simulink model "Battery_PowerEnergy_GridSOC_netz"  (R2024b)
settings: Solver=ode3  StartTime=0.0  StopTime=8759.75  FixedStep=10  RelTol=1e-3
model workspace (MAT data in the model file):
  Cc_tab = [1.5 1.55813461538 1.61558974359 1.67194230769 1.72676923077 1.7796474359 1.83015384615 1.87786538462 1.92235897436 1.96321153846 2 2.03486538462 2.07007692308 2.10540384615 2.14061538462 2.17548076923 2.20976923077 2.24325 2.27569230769 2.30686538462 2.33653846154 2.36448076923 2.39046153846 2.41425 2.43561538462 2.45432692308 2.47015384615 2.48286538462 2.49223076923 2.49801923077 2.5 2.49771933962 2.49109433962 2.4804504717 2.46611320755 2.44840801887 2.42766037736 2.40419575472 2.37833962264 2.35041745283 2.32075471698 2.28967688679 2.25750943396 2.22457783019 2.19120754717 2.1577240566 2.12445283019 2.09171933962 2.0598490566 2.02916745283 2 1.97106753319 1.94093774983 1.90970641509 1.8774692942 1.84432215234 1.81036075472 1.77568086653 1.74037825297 1.70454867925 1.66828791055 1.63169171209 1.59485584906 1.55787608665 1.52084819008 1.48386792453 1.44703105521 1.41043334731 1.37417056604 1.33833847659 1.30303284416 1.26834943396 1.23438401118 1.20123234102 1.16899018868 1.13775331936 1.10761749825 1.07867849057 1.0510320615 1.02477397624 1 0.97712 0.95616 0.93664 0.91808 0.9 0.88192 0.86336 0.84384 0.82288 0.8 0.77531 0.74928 0.72197 0.69344 0.66375 0.63296 0.60113 0.56832 0.53459 0]
  Cd_tab = [0 0.811245454545 0.824872727273 0.840718181818 0.858618181818 0.878409090909 0.899927272727 0.923009090909 0.947490909091 0.973209090909 1 1.02948863636 1.06318181818 1.10073863636 1.14181818182 1.18607954545 1.23318181818 1.28278409091 1.33454545455 1.388125 1.44318181818 1.499375 1.55636363636 1.61380681818 1.67136363636 1.72869318182 1.78545454545 1.84130681818 1.89590909091 1.94892045455 2 2.05044932432 2.1017027027 2.15361824324 2.20605405405 2.25886824324 2.31191891892 2.36506418919 2.41816216216 2.47107094595 2.52364864865 2.57575337838 2.62724324324 2.67797635135 2.72781081081 2.77660472973 2.82421621622 2.87050337838 2.91532432432 2.95853716216 3 3.04114214214 3.08337137137 3.12651351351 3.17039439439 3.21483983984 3.25967567568 3.30472772773 3.34982182182 3.39478378378 3.43943943944 3.48361461461 3.52713513514 3.56982682683 3.61151551552 3.65202702703 3.69118718719 3.72882182182 3.76475675676 3.79881781782 3.83083083083 3.86062162162 3.88801601602 3.91283983984 3.93491891892 3.95407907908 3.97014614615 3.98294594595 3.9923043043 3.99804704705 4 4 4 4 4 4 4 4 4 4 4 4 4 4 4 4 4 4 4 4 4]
  E_nom = 28200
  P_grid_max = 76000
  eta_c = 0.96
  eta_d = 0.96
  soc_bp = [0 0.01 0.02 0.03 0.04 0.05 0.06 0.07 0.08 0.09 0.1 0.11 0.12 0.13 0.14 0.15 0.16 0.17 0.18 0.19 0.2 0.21 0.22 0.23 0.24 0.25 0.26 0.27 0.28 0.29 0.3 0.31 0.32 0.33 0.34 0.35 0.36 0.37 0.38 0.39 0.4 0.41 0.42 0.43 0.44 0.45 0.46 0.47 0.48 0.49 0.5 0.51 0.52 0.53 0.54 0.55 0.56 0.57 0.58 0.59 0.6 0.61 0.62 0.63 0.64 0.65 0.66 0.67 0.68 0.69 0.7 0.71 0.72 0.73 0.74 0.75 0.76 0.77 0.78 0.79 0.8 0.81 0.82 0.83 0.84 0.85 0.86 0.87 0.88 0.89 0.9 0.91 0.92 0.93 0.94 0.95 0.96 0.97 0.98 0.99 1]
libraries: simulink x1
settings Model: Creator=Corbinian  LastModifiedBy=Corbinian
settings SolverCC: MaxConsecutiveMinStep=1000
settings DataIOCC: SignalLogging=off  ReturnWorkspaceOutputs=off

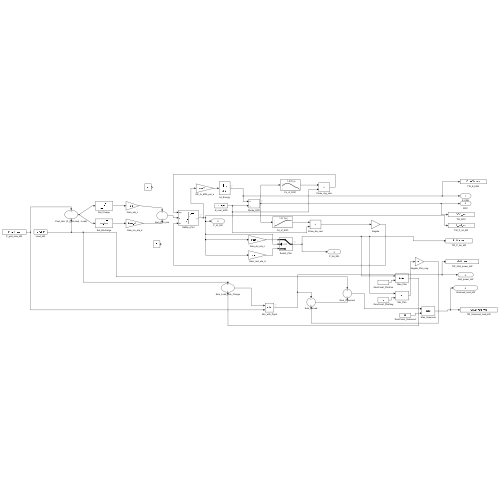
[thumbnail: Simulink's stored preview of the top-level diagram]
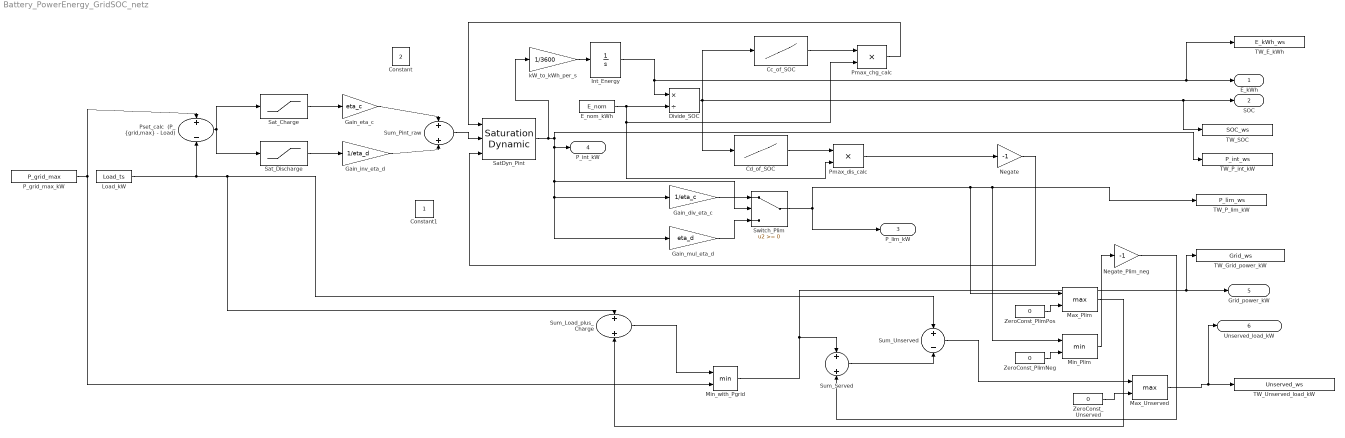
== system Battery_PowerEnergy_GridSOC_netz ==
  Cc_of_SOC : Lookup_n-D  NumberOfTableDimensions=1  BreakpointsForDimension1=soc_bp  Table=Cc_tab  InternalRulePriority=Speed  RndMeth=Simplest
  Cd_of_SOC : Lookup_n-D  NumberOfTableDimensions=1  BreakpointsForDimension1=soc_bp  Table=Cd_tab  InternalRulePriority=Speed  RndMeth=Simplest
  Constant : Constant  Value=2
  Constant1 : Constant
  Divide_SOC : Product  Inputs=*/
  E_nom_kWh : Constant  Value=E_nom
  Gain_div_eta_c : Gain  Gain=1/eta_c
  Gain_eta_c : Gain  Gain=eta_c
  Gain_inv_eta_d : Gain  Gain=1/eta_d
  Gain_mul_eta_d : Gain  Gain=eta_d
  Int_Energy : Integrator  InitialCondition=2000  LimitOutput=on  UpperSaturationLimit=E_nom  LowerSaturationLimit=0
  Load_kW : FromWorkspace  VariableName=Load_ts
  Max_Plim : MinMax  Function=max  Inputs=2
  Max_Unserved : MinMax  Function=max  Inputs=2
  Min_Plim : MinMax  Inputs=2
  Min_with_Pgrid : MinMax  Inputs=2
  Negate : Gain  Gain=-1
  Negate_Plim_neg : Gain  Gain=-1
  P_grid_max_kW : Constant  Value=P_grid_max
  Pmax_chg_calc : Product
  Pmax_dis_calc : Product
  "Pset_calc  (P_{grid,max} - Load)" : Sum  Inputs=+-
  SatDyn_Pint : simulink/Discontinuities/Saturation Dynamic  OutMin=[]  OutMax=[]  OutDataTypeStr=Inherit: Same as second input  OutDataType=fixdt(1, 16)  OutScaling=2^-10  DoSatur=off
  Sat_Charge : Saturate  UpperLimit=Inf  LowerLimit=0
  Sat_Discharge : Saturate  UpperLimit=0  LowerLimit=-Inf
  Sum_Load_plus_Charge : Sum
  Sum_Pint_raw : Sum
  Sum_Served : Sum
  Sum_Unserved : Sum  Inputs=+-
  Switch_Plim : Switch  SaturateOnIntegerOverflow=off  InputSameDT=off
  TW_E_kWh : ToWorkspace  VariableName=E_kWh_ws  SaveFormat=Structure With Time  SampleTime=-1
  TW_Grid_power_kW : ToWorkspace  VariableName=Grid_ws  SaveFormat=Structure With Time  SampleTime=-1
  TW_P_int_kW : ToWorkspace  VariableName=P_int_ws  SaveFormat=Structure With Time  SampleTime=-1
  TW_P_lim_kW : ToWorkspace  VariableName=P_lim_ws  SaveFormat=Structure With Time  SampleTime=-1
  TW_SOC : ToWorkspace  VariableName=SOC_ws  SaveFormat=Structure With Time  SampleTime=-1
  TW_Unserved_load_kW : ToWorkspace  VariableName=Unserved_ws  SaveFormat=Structure With Time  SampleTime=-1
  ZeroConst_PlimNeg : Constant  Value=0
  ZeroConst_PlimPos : Constant  Value=0
  ZeroConst_Unserved : Constant  Value=0
  kW_to_kWh_per_s : Gain  Gain=1/3600
  E_kWh : Outport
  SOC : Outport  Port=2
  P_lim_kW : Outport  Port=3
  P_int_kW : Outport  Port=4
  Grid_power_kW : Outport  Port=5
  Unserved_load_kW : Outport  Port=6
  wires:
  P_grid_max_kW/1 -> "Pset_calc  (P_{grid,max} - Load)"/1, Min_with_Pgrid/2
  Load_kW/1 -> "Pset_calc  (P_{grid,max} - Load)"/2, Sum_Load_plus_Charge/1, Sum_Unserved/1
  "Pset_calc  (P_{grid,max} - Load)"/1 -> Sat_Charge/1, Sat_Discharge/1
  Sat_Charge/1 -> Gain_eta_c/1
  Sat_Discharge/1 -> Gain_inv_eta_d/1
  Gain_eta_c/1 -> Sum_Pint_raw/1
  Gain_inv_eta_d/1 -> Sum_Pint_raw/2
  Int_Energy/1 -> Divide_SOC/1, TW_E_kWh/1, E_kWh/1
  E_nom_kWh/1 -> Pmax_chg_calc/2, Pmax_dis_calc/2, Divide_SOC/2
  Divide_SOC/1 -> Cd_of_SOC/1, TW_SOC/1, SOC/1, Cc_of_SOC/1
  Cc_of_SOC/1 -> Pmax_chg_calc/1
  Cd_of_SOC/1 -> Pmax_dis_calc/1
  Pmax_chg_calc/1 -> SatDyn_Pint/1
  Pmax_dis_calc/1 -> Negate/1
  Negate/1 -> SatDyn_Pint/3
  SatDyn_Pint/1 -> Gain_mul_eta_d/1, Gain_div_eta_c/1, Switch_Plim/2, P_int_kW/1, TW_P_int_kW/1, kW_to_kWh_per_s/1
  kW_to_kWh_per_s/1 -> Int_Energy/1
  Gain_div_eta_c/1 -> Switch_Plim/1
  Gain_mul_eta_d/1 -> Switch_Plim/3
  Switch_Plim/1 -> Max_Plim/1, Min_Plim/1, TW_P_lim_kW/1, P_lim_kW/1
  Sum_Load_plus_Charge/1 -> Min_with_Pgrid/1
  Min_with_Pgrid/1 -> TW_Grid_power_kW/1, Grid_power_kW/1, Sum_Served/1
  Negate_Plim_neg/1 -> Sum_Served/2
  Sum_Served/1 -> Sum_Unserved/2
  Sum_Pint_raw/1 -> SatDyn_Pint/2
  ZeroConst_Unserved/1 -> Max_Unserved/2
  ZeroConst_PlimPos/1 -> Max_Plim/2
  ZeroConst_PlimNeg/1 -> Min_Plim/2
  Max_Unserved/1 -> Unserved_load_kW/1, TW_Unserved_load_kW/1
  Sum_Unserved/1 -> Max_Unserved/1
  Max_Plim/1 -> Sum_Load_plus_Charge/2
  Min_Plim/1 -> Negate_Plim_neg/1
